simulink model "EV6_LUT_FourWheel_EV6Battery77p4kWh_PowerCorrected"  (R2024a)
settings: Solver=ode4  StartTime=0  StopTime=60  FixedStep=0.001  RelTol=1e-3
PreLoadFcn:
  | VSS_BICYCLE=Simulink.Variant('Dual=0');
  | VSS_DUAL=Simulink.Variant('Dual=1');
  | Dual=1;
  | load('DriveCycle2.mat')
PostLoadFcn:
  | if any(exist('dsrtsu_mdlpostloadfcn', 'file') ~= 0), dsrtsu_mdlpostloadfcn('Execute', bdroot); end
InitFcn:
  | , if any(exist('rtifpga_mdlclblib', 'file') ~= 0), rtifpga_mdlclblib('Init', bdroot); end,
  | , if any(exist('dsmpb_private', 'file') ~= 0), dsmpb_private('dsmpb_mdlclblib', 'Init', bdroot); end,
  | load('DriveCycle2.mat')
model workspace (MAT data in the model file):
  DiffRatio = 10.65
  EV6_2023_BattBranchCapacity_Ah = 55.5236728838
  EV6_2023_BattEnergy_kWh = 77.4
  EV6_2023_BattNominalVoltage_V = 697
  EV6_2023_BattNumCellsParallel = 2
  EV6_2023_BattNumCellsSeries = 192
  EV6_2023_BattOpenVoltCapBpts = [0 0.1 0.2 0.3 0.4 0.5 0.6 0.7 0.8 0.9 1]
  EV6_2023_BattOpenVoltTbl = [2.96762142548 3.40364281191 3.47417488548 3.54470541822 3.61523441014 3.68576186124 3.75628777151 3.82681214095 3.94527005036 4.07101207308 4.2120755254]
  EV6_2023_BattPackCapacity_Ah = 111.047345768
  EV6_2023_BattResistSocBpts = [0 0.2 0.4 0.6 0.8 1]
  EV6_2023_BattResistTbl = [0.0163620057716 0.0118174152018 0.00807187352333 0.00375663957972 0.00266904525531 0.00103635901355 0.0019014404175 0.0172368903217 0.0121226074867 0.00758541551769 0.00474065349228 0.00337561163613 ... (42 elements, 7x6)]
  EV6_2023_BattResistTempBpts = [243.1 253.1 263.1 273.1 283.1 298.1 313.1]
  EV6_2023_InitialPackOCV_V = 726.471714233
  EV6_2023_InitialSOC = 0.638878863672
  EV6_BattCellCapacity_Ah = 60.3
  EV6_BattInitialSOC = 0.638878863672
  EV6_BattOCV_Cell_V = [2.96762142548 3.40364281191 3.47417488548 3.54470541822 3.61523441014 3.68576186124 3.75628777151 3.82681214095 3.94527005036 4.07101207308 4.2120755254]
  EV6_BattOCV_SOC = [0 0.1 0.2 0.3 0.4 0.5 0.6 0.7 0.8 0.9 1]
  EV6_BattPackCapacity_Ah = 120.6
  EV6_BattParallelCells = 2
  EV6_BattResistanceSOC = [0 0.2 0.4 0.6 0.8 1]
  EV6_BattResistanceTable_Ohm = [0.0163620057716 0.0118174152018 0.00807187352333 0.00375663957972 0.00266904525531 0.00103635901355 0.0019014404175 0.0172368903217 0.0121226074867 0.00758541551769 0.00474065349228 0.00337561163613 ... (42 elements, 7x6)]
  EV6_BattResistanceTemp_K = [243.1 253.1 263.1 273.1 283.1 298.1 313.1]
  EV6_BattSeriesCells = 192
  EV6_FinalDriveRatio = 10.65
  EV6_TargetPackResistance_Ohm = 0.132763804608
  Gas = 0.383333333333
undefined symbols (not defined in the file): accel_bp_mps2, AccelCmd, ActTqLF_Nm_, ActTqLR_Nm_, ActTqRF_Nm_, ActTqRR_Nm_, BattChargeLimitMaxPwr, BattChargeLimitSocBpts, BattChargeLimitTbl, BattDischargeLimitSocBpts, BattDischargeLimitTbl, BattDischargeMaxPwr, BrakeMaxPrs, BrakeMaxTrq, ChassisDistCg2FrontAxle, ChassisDistCg2RearAxle, ChassisVehMass, CltchCmd, CoastDown, DecelCmd, DiscIntNeverNeededParam, EnvGravCnst, EnvPrs, EnvTemp, EV6_RegenTorqueGain, EV6_TractionTorqueGain, front_share_regen_3d, front_share_traction_3d, FuelSpecificGrav, GearCmd, h, InitStates, lgSw, limitedMCT, MCT, MtrEffSpdBpts, MtrEffTbl, MtrEffTrqBpts, MtrPwrMax, MtrTrqMax, out_1, pMCT, RealSimPara, Ref_speed, Ref_time, regen_torque_bp_Nm, speed_bp_kph, SteeringCmd, SupvsryCtrlRegenBrkCutOffTbl, SupvsryCtrlRegenSpdBpts, TestScnrioCycleNum, traction_torque_bp_Nm, US06, VEH
libraries: VSIGenLib x65, simulink x54, etargetslib x38, dsmpblib x24, vehdynlibtire x12, autolibshared x11, vehdynlibsuspension x7, vehdynlibtirecommon x7, autolibpowerinfoutils x6, autolibutils x5, autolibsharedcoupling x4, autolibmappedmotor x4
(part 19 of 19)

== stateflow chart EV6_LUT_FourWheel_EV6Battery77p4kWh_PowerCorrected/Vehicle Under Test1/Vehicle/Rototest and ORNL Interface/To Rototest with Band-Aid/Band-Aid/Band-Aid ==
  state dStop
    en:
    OutMode = 0;
    State = 3;
  state Running
    state SpeedMode
      en:
      OutMode = 1;
      state Blend
        en:
        OutSpd = InSpd;
        State = 0.1;
      state Driving
        du:
        OutSpd = InSpd;
        State = 0.2;
      (default) -> Blend
      Blend -> Driving
    state TorqueMode
      en:
      OutMode = 0;
      du:
      State = 1;
    (default) -> SpeedMode
    TorqueMode -> Blend : [after(SettleTime, sec) || ...
        | ~BrkSw]
    SpeedMode -> TorqueMode : [(any(InSpd < SpdLatchThr) && ...
        | (VehSpd_kph < VehSpdThr_kph) && BrkSw)]
  note: The vehicle will enter speed mode (driving) if:
      | The vehicle has been in torque mode for a calibrated time (settleTime) AND
      | The Input Speed (InSpd) is greater than a Launch Treshold (LaunchSpdThr) OR
      | The Input Torque (InTrq) is greater than calibrated torque value (LaunchTrqThr).
      | Criteria 1) sees the dyno has "settled" and allows the dyno to go back into speed mode.
      | Criteria 2) sees the vehicle is attempting to reaccelerate and pushes into speed mode.
      |
      | The vehicle will enter torque mode (zero) if:
      | Input Speed (InSpd) goes below the calibrated speed (SpdLatchThr) AND
      | Brake (BrkSw) is active.
      | 2) dStop is activated.
      | Criteria 1) sees the vehicle is attempting to come to a stop and unloads the dyno.
      | Criteria 2) is SHTF.
      |
      | && ...
      | (InSpd > LaunchSpdThr || ...
      | InTrq > LaunchTrqThr)
  (default) -> dStop
  Running -> dStop : [dStop]
  dStop -> Running : [~dStop]
  data: LaunchSpdThr input; LaunchTrqThr input; SpdLatchThr input; BrkSw input; InSpd input; InTrq input; OutMode output size=1; OutSpd output; State output; SettleTime input; dStop input; VehSpd_kph input; VehSpdThr_kph input

== matlab function EV6_LUT_FourWheel_EV6Battery77p4kWh_PowerCorrected/Vehicle Under Test1/Vehicle/Rototest and ORNL Interface/To Rototest with Band-Aid/RotoTestEthTx/MATLAB Function ==
  data: SpTqRR input; y output; SpTqLR input; SpTqRF input; SpTqLF input; SystemActive input
function y = fcn(SpTqRR, SpTqLR, SpTqRF, SpTqLF, SystemActive)

y = 0;
if SpTqRR == 1 && SystemActive == 0
    y = 30;
elseif SpTqRR == 0 && SystemActive == 0
    y = 0;
elseif SpTqRR == 1 && SystemActive == 1
    y = 31;
elseif SpTqRR == 0 && SystemActive == 1
    y = 1;
end

y = uint8(y);

== matlab function EV6_LUT_FourWheel_EV6Battery77p4kWh_PowerCorrected/Vehicle Under Test1/Vehicle/Vehicle Dynamics/Vehicle 14DOF/Wheels and Tires/VDBS/Tires/MF Tires/MATLAB Function ==
  data: axleTorq input; switchFlag output; wheelSpd input
function switchFlag = fcn(axleTorq, wheelSpd)

% if braking and vehicle has stopped
%if (abs(axleTorq) < 1e-5 && abs(wheelSpd) < 1e-5)
if abs(wheelSpd) < 1e-5
    switchFlag = 1;
else
    switchFlag = 0;
end

== matlab function EV6_LUT_FourWheel_EV6Battery77p4kWh_PowerCorrected/Vehicle Under Test1/Vehicle/Vehicle Dynamics/Vehicle 14DOF/Wheels and Tires/VDBS/Tires/MF Tires/MATLAB Function1 ==
  data: axleTorq input; switchFlag output; wheelSpd input
function switchFlag = fcn(axleTorq, wheelSpd)

% if braking and vehicle has stopped
%if (abs(axleTorq) < 1e-5 && abs(wheelSpd) < 1e-5)
if abs(wheelSpd) < 1e-5
    switchFlag = 1;
else
    switchFlag = 0;
end

== matlab function EV6_LUT_FourWheel_EV6Battery77p4kWh_PowerCorrected/Vehicle Under Test1/Vehicle/Vehicle Dynamics/Vehicle 14DOF/Wheels and Tires/VDBS/Tires/MF Tires/MATLAB Function2 ==
  data: axleTorq input; switchFlag output; wheelSpd input
function switchFlag = fcn(axleTorq, wheelSpd)

% if braking and vehicle has stopped
%if (abs(axleTorq) < 1e-5 && abs(wheelSpd) < 1e-5)
if abs(wheelSpd) < 1e-5
    switchFlag = 1;
else
    switchFlag = 0;
end

== matlab function EV6_LUT_FourWheel_EV6Battery77p4kWh_PowerCorrected/Vehicle Under Test1/Vehicle/Vehicle Dynamics/Vehicle 14DOF/Wheels and Tires/VDBS/Tires/MF Tires/MATLAB Function3 ==
  data: axleTorq input; switchFlag output; wheelSpd input
function switchFlag = fcn(axleTorq, wheelSpd)

% if braking and vehicle has stopped
%if (abs(axleTorq) < 1e-5 && abs(wheelSpd) < 1e-5)
if abs(wheelSpd) < 1e-5
    switchFlag = 1;
else
    switchFlag = 0;
end

== matlab function EV6_LUT_FourWheel_EV6Battery77p4kWh_PowerCorrected/Vehicle Under Test1/Vehicle/Vehicle Dynamics/Vehicle 7DOF/For 3D Visualization ==
  data: angles output size=3; angleIn input size=3; GeomXYZ output size=3; GemoXYZIn input size=3; GroundZ input size=4; trackW parameter; wheelB parameter
function [angles,GeomXYZ]= three26(angleIn, GemoXYZIn, GroundZ,trackW, wheelB)%#codegen
coder.allowpcode('plain')
% Copyright 2018 The MathWorks, Inc.
[angles,GeomXYZ]= vdynthree2six(angleIn, GemoXYZIn, GroundZ,trackW, wheelB);
